simulink model "My_gfm_pv_plus_sil_motor"  (R2018b)
settings: Solver=ode45  StartTime=0.0  StopTime=22  RelTol=1e-3
PreLoadFcn:
  | lmodelDir = fileparts(get_param(bdroot,'FileName'));
  | 
  | load_system(fullfile(modelDir,'controls_element_lib.slx'));
  | load_system(fullfile(modelDir,'test_sequence_lib.slx'));
InitFcn:
  | close all;
  | clear all;
  | clc;
  | 
  | % frequency nominals
  | F_NOM = 60;
  | W_NOM = 2 * pi * F_NOM;
  | 
  | C_DC = 0.4; % Supercap: 0.5sec * 5MW
  | V_LVDC_NOM = 1000;
  | 
  | % base values relative to inverter
  | % --------------------------------
  | VLL_INV_NOM = 480;
  | P_INV_NOM = 1e6;
  | Q_INV_NOM = 0.5e6;
  | S_INV_NOM = sqrt(P_INV_NOM^2 + Q_INV_NOM^2);
  | 
  | I_INV_BASE = S_INV_NOM/(sqrt(3)*VLL_INV_NOM);
  | Z_INV_BASE = VLL_INV_NOM^2/S_INV_NOM;
  | L_INV_BASE = Z_INV_BASE / W_NOM;
  | C_INV_BASE = 1 / (Z_INV_BASE * W_NOM);
  | 
  | % nominal ratings for power system model
  | % --------------------------------------
  | INVERTER_COUNT = 100;
  | 
  | VLV_NOM = VLL_INV_NOM;
  | VMV_NOM = 35e3;
  | VHV_NOM = 230e3;
  | S_PLANT = INVERTER_COUNT * S_INV_NOM;
  | 
  | N_GSU = VHV_NOM/VMV_NOM;
  | N_MVT = VMV_NOM/VLV_NOM;
  | 
  | I_LV_BASE = S_PLANT/(sqrt(3)*VLV_NOM);
  | I_MV_BASE = S_PLANT/(sqrt(3)*VMV_NOM);
  | I_HV_BASE = S_PLANT/(sqrt(3)*VHV_NOM);
  | 
  | Z_LV_BASE = VLV_NOM^2/S_PLANT;
  | Z_MV_BASE = VMV_NOM^2/S_PLANT;
  | Z_HV_BASE = VHV_NOM^2/S_PLANT;
  | 
  | L_LV_BASE = Z_LV_BASE / W_NOM;
  | L_MV_BASE = Z_MV_BASE / W_NOM;
  | L_HV_BASE = Z_HV_BASE / W_NOM;
  | C_LV_BASE = 1 / (Z_LV_BASE * W_NOM);
  | C_MV_BASE = 1 / (Z_MV_BASE * W_NOM);
  | C_HV_BASE = 1 / (Z_HV_BASE * W_NOM);
  | 
  | %---------------------------------------
  | %Motor Control
  | 
  | Jsys = 20;
  | Fpu = 0.02;
  | MtrPwr = 500000 ;
  | MtrFreq = 60;
  | MtrPp = 2;
  | MtrWm = 2 * pi *MtrFreq/MtrPp;
  | MtrTrq = MtrPwr / MtrWm;
  | F = (Fpu*MtrTrq)/MtrWm;
  | 
  | SpeedBW = 2 * pi * 0.5;
  | Zeta = 1;
  | H = (0.5 * Jsys * MtrWm^2)/MtrPwr;
  | Kpv = SpeedBW * (H * 2) * 2 * Zeta;
  | Kiv = (SpeedBW^2) * (H * 2) * 1;
undefined symbols (not defined in the file): MtrNpFreq, MtrNpTrq, Pp, Ts_Control_1
libraries: test_sequence_lib x13, controls_element_lib x8, simulink x6
settings Model: SimulationMode=accelerator  Creator=halatrash  LastModifiedBy=ahhei
settings SolverCC: ZeroCrossAlgorithm=Adaptive
settings DataIOCC: ReturnWorkspaceOutputs=on
settings DebuggingCC: MaxConsecutiveZCsMsg=warning  IgnoredZcDiagnostic=none  UnconnectedInputMsg=none  UnconnectedOutputMsg=none  UnconnectedLineMsg=none
settings ModelReferenceCC: EnableRefExpFcnMdlSchedulingChecks=off
settings RTWCC: Description=Generic Real-Time Target

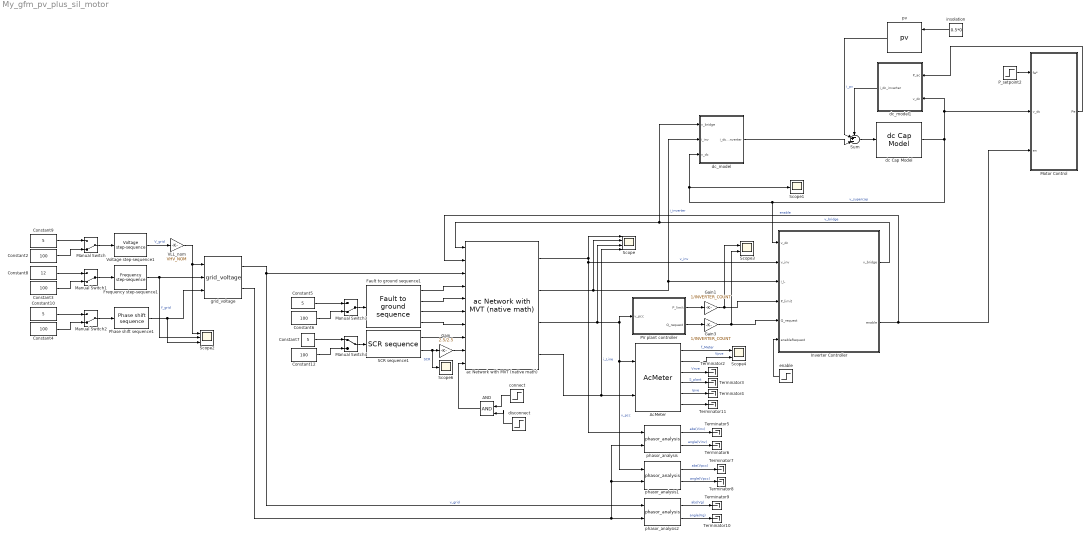
== system My_gfm_pv_plus_sil_motor ==
  AND : Logic  IconShape=distinctive  AllPortsSameDT=off  OutDataTypeStr=boolean
  AcMeter : test_sequence_lib/AcMeter  VllRated=VHV_NOM
  Constant{5,7,9..10} (4 alike) : Constant  Value=5
  Constant{2..4,6,12} (5 alike) : Constant  Value=100
  Constant8 : Constant  Value=12
  Fault to ground sequence1 : test_sequence_lib/Fault to ground sequence  SystemSampleTime=-1
  Frequency step-sequence1 : test_sequence_lib/Frequency step-sequence  SystemSampleTime=-1
  Gain : Gain  Gain=2.5/2.5
  Gain1 : Gain  Gain=1/INVERTER_COUNT
  Gain3 : Gain  Gain=1/INVERTER_COUNT
  Inverter Controller : Subsystem
  Manual Switch{,1..3} (4 alike) : ManualSwitch  CurrentSetting=0
  Manual Switch4 : ManualSwitch
  Motor Control : Subsystem
  PV plant controller : Subsystem  AncestorBlock=controls_element_lib/PV plant controller
  P_setpoint2 : Step  Time=4  SampleTime=0
  Phase shift sequence1 : test_sequence_lib/Phase shift sequence  SystemSampleTime=-1
  SCR sequence1 : test_sequence_lib/SCR sequence  SystemSampleTime=-1
  Scope : Scope  NumInputPorts=4
  Scope1 : Scope
  Scope2 : Scope  NumInputPorts=3
  Scope3 : Scope  NumInputPorts=2
  Scope4 : Scope  NumInputPorts=2
  Scope6 : Scope
  Sum : Sum  Inputs=-+-|
  Terminator{2..11} (10 alike) : Terminator
  VLL_nom : Gain  Gain=VHV_NOM
  Voltage step-sequence1 : test_sequence_lib/Voltage step-sequence  SystemSampleTime=-1
  ac Network with MVT (native math) : test_sequence_lib/ac Network with MVT (native math)  SystemSampleTime=-1
  connect : Step  Time=0  SampleTime=0
  dc Cap Model : test_sequence_lib/dc Cap Model  SystemSampleTime=-1
  dc_model : Subsystem  AncestorBlock=test_sequence_lib/dc_model
  dc_model1 : Subsystem  AncestorBlock=test_sequence_lib/dc_model
  disconnect : Step  Time=97  Before=1  After=0  SampleTime=0
  enable : Step  Time=2  SampleTime=0
  grid_voltage : test_sequence_lib/grid_voltage  SystemSampleTime=-1
  insolation : Constant  Value=0.5*0
  phasor_analysis : test_sequence_lib/phasor_analysis  SystemSampleTime=-1
  phasor_analysis1 : test_sequence_lib/phasor_analysis  SystemSampleTime=-1
  phasor_analysis2 : test_sequence_lib/phasor_analysis  SystemSampleTime=-1
  pv : test_sequence_lib/pv  VopenCircuit=1500  IshortCircuit=1000
  wires:
  ac Network with MVT (native math)/3 -> Scope/3, PV plant controller/1(v_pcc), phasor_analysis1/1, AcMeter/1  "v_pcc"
  Gain3/1 -> Scope3/2, Inverter Controller/5(Q_request)
  AcMeter/2 -> Scope4/2  "Vpve"
  phasor_analysis2/2 -> Terminator10/1  "angle(Vg)"
  phasor_analysis1/2 -> Terminator8/1  "angle(Vpcc)"
  AcMeter/5 -> Terminator4/1  "Ipve"
  phasor_analysis2/1 -> Terminator9/1  "abs(Vg)"
  Inverter Controller/1(v_bridge) -> ac Network with MVT (native math)/1, dc_model/1(v_bridge)  "v_bridge"
  phasor_analysis1/1 -> Terminator7/1  "abs(Vpcc)"
  grid_voltage/1 -> ac Network with MVT (native math)/3, phasor_analysis2/1  "v_grid"
  connect/1 -> AND/1
  dc Cap Model/1 -> dc_model1/2(v_dc), Motor Control/2(v_dc), Scope1/1, dc_model/3(v_dc), Inverter Controller/1(v_dc)  "v_supercap"
  AcMeter/4 -> Terminator3/1  "S_plant"
  Phase shift sequence1/1 -> Scope2/3, grid_voltage/3
  Frequency step-sequence1/1 -> Scope2/2, grid_voltage/2  "f_grid"
  phasor_analysis/1 -> Terminator5/1  "abs(Vinv)"
  AcMeter/3 -> Terminator2/1  "Vnve"
  phasor_analysis/2 -> Terminator6/1  "angle(Vinv)"
  Sum/1 -> dc Cap Model/1
  ac Network with MVT (native math)/1 -> Scope/1, Inverter Controller/2(v_inv), phasor_analysis/1  "v_inv"
  AND/1 -> ac Network with MVT (native math)/10
  AcMeter/6 -> Terminator11/1
  Voltage step-sequence1/1 -> VLL_nom/1  "V_grid"
  grid_voltage/2 -> phasor_analysis1/2, phasor_analysis/2, phasor_analysis2/2
  disconnect/1 -> AND/2
  ac Network with MVT (native math)/2 -> Scope/2, Inverter Controller/3(i_L), dc_model/2(i_inv)  "i_inverter"
  PV plant controller/2(Q_request) -> Gain3/1
  ac Network with MVT (native math)/4 -> Scope/4, AcMeter/2  "i_Line"
  dc_model/1(i_dc_inverter) -> Sum/3
  Inverter Controller/2(enable) -> Motor Control/3(en), ac Network with MVT (native math)/2  "enable"
  VLL_nom/1 -> Scope2/1, grid_voltage/1
  enable/1 -> Inverter Controller/6(enableRequest)
  insolation/1 -> pv/1
  pv/1 -> Sum/2  "i_pv"
  PV plant controller/1(P_limit) -> Gain1/1
  Gain1/1 -> Scope3/1, Inverter Controller/4(P_limit)
  AcMeter/1 -> Scope4/1  "f_Meter"
  Constant10/1 -> Manual Switch2/1
  Constant9/1 -> Manual Switch/1
  Constant4/1 -> Manual Switch2/2
  Constant8/1 -> Manual Switch1/1
  Manual Switch1/1 -> Frequency step-sequence1/1
  Manual Switch2/1 -> Phase shift sequence1/1
  Manual Switch/1 -> Voltage step-sequence1/1
  Constant3/1 -> Manual Switch1/2
  Constant2/1 -> Manual Switch/2
  Constant12/1 -> Manual Switch4/2
  Constant6/1 -> Manual Switch3/2
  Manual Switch4/1 -> SCR sequence1/1
  Constant5/1 -> Manual Switch3/1
  Manual Switch3/1 -> Fault to ground sequence1/1
  Fault to ground sequence1/4 -> ac Network with MVT (native math)/7
  SCR sequence1/2 -> Scope6/1, Gain/1  "SCR"
  Fault to ground sequence1/1 -> ac Network with MVT (native math)/4
  SCR sequence1/1 -> ac Network with MVT (native math)/8
  Constant7/1 -> Manual Switch4/1
  Fault to ground sequence1/3 -> ac Network with MVT (native math)/6
  Fault to ground sequence1/2 -> ac Network with MVT (native math)/5
  Gain/1 -> ac Network with MVT (native math)/9
  P_setpoint2/1 -> Motor Control/1(fe*)
  Motor Control/1(Pe) -> dc_model1/1(P_ac)
  dc_model1/1(i_dc_inverter) -> Sum/1

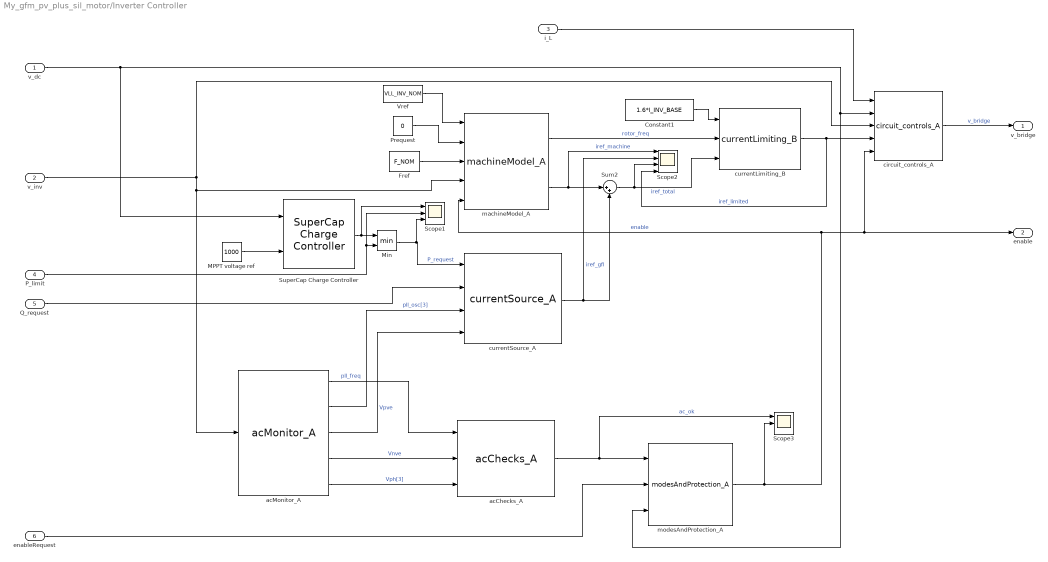
== system My_gfm_pv_plus_sil_motor/Inverter Controller ==
  v_dc : Inport
  v_inv : Inport  Port=2
  i_L : Inport  Port=3
  P_limit : Inport  Port=4
  Q_request : Inport  Port=5
  enableRequest : Inport  Port=6
  Constant1 : Constant  Value=1.6*I_INV_BASE
  Fref : Constant  Value=F_NOM
  MPPT voltage ref : Constant  Value=1000
  Min : MinMax  Inputs=2
  Prequest : Constant  Value=0
  Scope1 : Scope  NumInputPorts=3
  Scope2 : Scope  NumInputPorts=4
  Scope3 : Scope  NumInputPorts=3
  Sum2 : Sum  Inputs=|++
  SuperCap Charge Controller : controls_element_lib/SuperCap Charge Controller  SystemSampleTime=-1
  Vref : Constant  Value=VLL_INV_NOM
  acChecks_A : controls_element_lib/acChecks_A  VllRated=VLL_INV_NOM  nominalFrequency=F_NOM  tRequalify=2  T_CNTL=1e-3
  acMonitor_A : controls_element_lib/acMonitor_A  VllRated=VLL_INV_NOM  nominalFrequency=F_NOM
  circuit_controls_A : controls_element_lib/circuit_controls_A  SystemSampleTime=-1
  currentLimiting_B : controls_element_lib/currentLimiting_B  IRated=I_INV_BASE  peakSoftLimit=2.6  peakHardLimit=3.6
  currentSource_A : controls_element_lib/currentSource_A  VllRated=VLL_INV_NOM  SRated=S_INV_NOM  nominalFrequency=F_NOM  Plimit=P_INV_NOM/S_INV_NOM  Qlimit=Q_INV_NOM/S_INV_NOM
  machineModel_A : controls_element_lib/machineModel_A  SRated=S_INV_NOM  VllRated=VLL_INV_NOM  nominalFrequency=F_NOM  inertialConstant=0.1  kDroop=0  kDamper=0.5  Xs=0.3  rs=0.08  Qlimit=0.5  wExciter=10
  modesAndProtection_A : controls_element_lib/modesAndProtection_A  dcOvervotlageThreshold=1800  dcUndervotlageThreshold=700  dcTripClearTimeout=0.2
  v_bridge : Outport  VectorParamsAs1DForOutWhenUnconnected=on
  enable : Outport  Port=2  VectorParamsAs1DForOutWhenUnconnected=on
  wires:
  Vref/1 -> machineModel_A/1
  Prequest/1 -> machineModel_A/2
  Fref/1 -> machineModel_A/3
  machineModel_A/2 -> Scope2/1, Sum2/1  "iref_machine"
  currentLimiting_B/1 -> Scope2/4, circuit_controls_A/4  "iref_limited"
  v_inv/1 -> circuit_controls_A/3, acMonitor_A/1, machineModel_A/4
  currentSource_A/1 -> Scope2/2, Sum2/2  "iref_gfl"
  Sum2/1 -> Scope2/3, currentLimiting_B/3  "iref_total"
  acMonitor_A/2 -> currentSource_A/3  "pll_osc[3]"
  Q_request/1 -> currentSource_A/2
  acMonitor_A/4 -> acChecks_A/2  "Vnve"
  enableRequest/1 -> modesAndProtection_A/2
  modesAndProtection_A/1 -> Scope3/2, machineModel_A/5, circuit_controls_A/5, enable/1  "enable"
  Min/1 -> Scope1/3, currentSource_A/1  "P_request"
  acMonitor_A/3 -> currentSource_A/4  "Vpve"
  Constant1/1 -> currentLimiting_B/1
  acMonitor_A/5 -> acChecks_A/3  "Vph[3]"
  acChecks_A/1 -> Scope3/1, modesAndProtection_A/1  "ac_ok"
  acMonitor_A/1 -> acChecks_A/1  "pll_freq"
  circuit_controls_A/1 -> v_bridge/1  "v_bridge"
  v_dc/1 -> modesAndProtection_A/3, circuit_controls_A/2, SuperCap Charge Controller/1
  i_L/1 -> circuit_controls_A/1
  machineModel_A/1 -> currentLimiting_B/2  "rotor_freq"
  MPPT voltage ref/1 -> SuperCap Charge Controller/2
  SuperCap Charge Controller/1 -> Scope1/1, Min/1
  P_limit/1 -> Scope1/2, Min/2

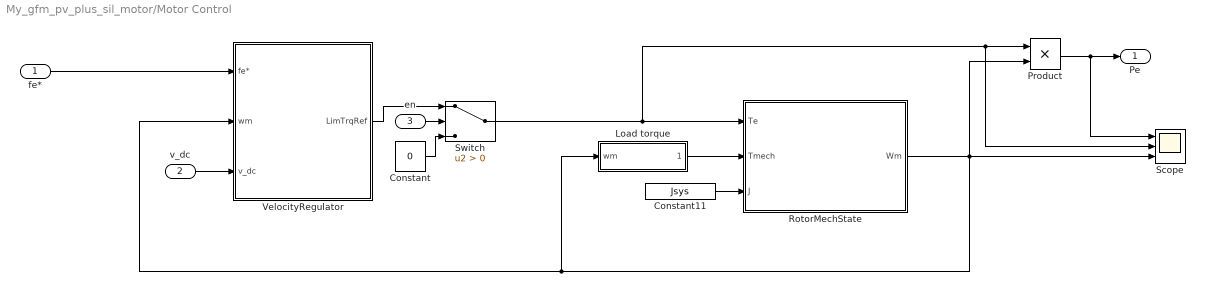
== system My_gfm_pv_plus_sil_motor/Motor Control ==
  fe* : Inport
  v_dc : Inport  Port=2
  en : Inport  Port=3
  Constant : Constant  Value=0
  Constant11 : Constant  Value=Jsys  OutDataTypeStr=double
  Load torque : Subsystem
  Product : Product
  RotorMechState : Subsystem
  Scope : Scope  NumInputPorts=3
  Switch : Switch  Criteria=u2 > Threshold
  VelocityRegulator : Subsystem
  Pe : Outport
  wires:
  RotorMechState/1(Wm) -> Product/2, Scope/3, VelocityRegulator/2(wm), Load torque/1(wm)
  Switch/1 -> Scope/2, Product/1, RotorMechState/1(Te)
  Constant11/1 -> RotorMechState/3(J)
  Load torque/1(" ") -> RotorMechState/2(Tmech)
  fe*/1 -> VelocityRegulator/1(fe*)
  Product/1 -> Scope/1, Pe/1
  v_dc/1 -> VelocityRegulator/3(v_dc)
  en/1 -> Switch/2
  VelocityRegulator/1(LimTrqRef) -> Switch/1
  Constant/1 -> Switch/3

== system My_gfm_pv_plus_sil_motor/PV plant controller ==
  v_pcc : Inport
  Frequency foldback : Subsystem
  Gain1 : Gain  Gain=S_PLANT
  Gain2 : Gain  Gain=S_PLANT
  Gain4 : Gain  Gain=1/VHV_NOM
  Meter : Subsystem
  VoltVAr : Subsystem
  P_limit : Outport  VectorParamsAs1DForOutWhenUnconnected=on
  Q_request : Outport  Port=2  VectorParamsAs1DForOutWhenUnconnected=on
  wires:
  Gain2/1 -> P_limit/1  "P_limit"
  Frequency foldback/1(limit_pu) -> Gain2/1
  Meter/1(f) -> Frequency foldback/1(f)
  v_pcc/1 -> Gain4/1
  Gain1/1 -> Q_request/1  "Q_request"
  Meter/2(V_estimate) -> VoltVAr/1(V)  "V_pu_plant"
  Gain4/1 -> Meter/1(v)
  VoltVAr/1(Q) -> Gain1/1

== system My_gfm_pv_plus_sil_motor/dc_model ==
  v_bridge : Inport
  i_inv : Inport  Port=2
  v_dc : Inport  Port=3
  Product : Product
  Product1 : Product  Inputs=*/
  Saturation : Saturate  UpperLimit=inf  LowerLimit=10
  Sum of Elements : Sum  Inputs=+
  i_dc_inverter : Outport  VectorParamsAs1DForOutWhenUnconnected=on
  wires:
  Saturation/1 -> Product1/2
  v_bridge/1 -> Product/1
  Product1/1 -> i_dc_inverter/1  "i_dc_inverter"
  Product/1 -> Sum of Elements/1
  i_inv/1 -> Product/2
  Sum of Elements/1 -> Product1/1  "P_ac"
  v_dc/1 -> Saturation/1

== system My_gfm_pv_plus_sil_motor/dc_model1 ==
  P_ac : Inport
  v_dc : Inport  Port=2
  Product1 : Product  Inputs=*/
  Saturation : Saturate  UpperLimit=inf  LowerLimit=10
  i_dc_inverter : Outport  VectorParamsAs1DForOutWhenUnconnected=on
  wires:
  Saturation/1 -> Product1/2
  Product1/1 -> i_dc_inverter/1
  P_ac/1 -> Product1/1
  v_dc/1 -> Saturation/1

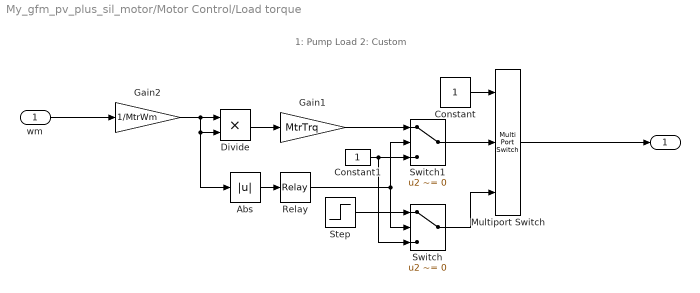
== system My_gfm_pv_plus_sil_motor/Motor Control/Load torque ==
  note: 1: Pump Load
      | 2: Custom
  wm : Inport
  Abs : Abs
  Constant : Constant
  Constant1 : Constant  OutDataTypeStr=single
  Divide : Product  Inputs=**
  Gain1 : Gain  Gain=MtrTrq
  Gain2 : Gain  Gain=1/MtrWm
  Multiport Switch : MultiPortSwitch  Inputs=2
  Relay : Relay  OnSwitchValue=0.01  OffSwitchValue=0.001
  Step : Step  Time=3  After=0.5*MtrTrq  SampleTime=0
  Switch : Switch  Criteria=u2 ~= 0
  Switch1 : Switch  Criteria=u2 ~= 0
  " " : Outport
  wires:
  Step/1 -> Switch/1
  Gain1/1 -> Switch1/1
  Constant/1 -> Multiport Switch/1
  Divide/1 -> Gain1/1
  wm/1 -> Gain2/1
  Switch/1 -> Multiport Switch/3
  Switch1/1 -> Multiport Switch/2
  Constant1/1 -> Switch/3, Switch1/3
  Relay/1 -> Switch1/2, Switch/2
  Abs/1 -> Relay/1
  Gain2/1 -> Abs/1, Divide/2, Divide/1
  Multiport Switch/1 -> " "/1

== system My_gfm_pv_plus_sil_motor/Motor Control/RotorMechState ==
  Te : Inport
  Tmech : Inport  Port=2
  J : Inport  Port=3
  Divide : Product  Inputs=*/
  Gain : Gain  Gain=F
  Integrator : Integrator
  Subtract : Sum  Inputs=-+-
  Wm : Outport
  wires:
  Te/1 -> Subtract/2
  Tmech/1 -> Subtract/3
  Subtract/1 -> Divide/1
  J/1 -> Divide/2
  Divide/1 -> Integrator/1
  Integrator/1 -> Gain/1, Wm/1
  Gain/1 -> Subtract/1

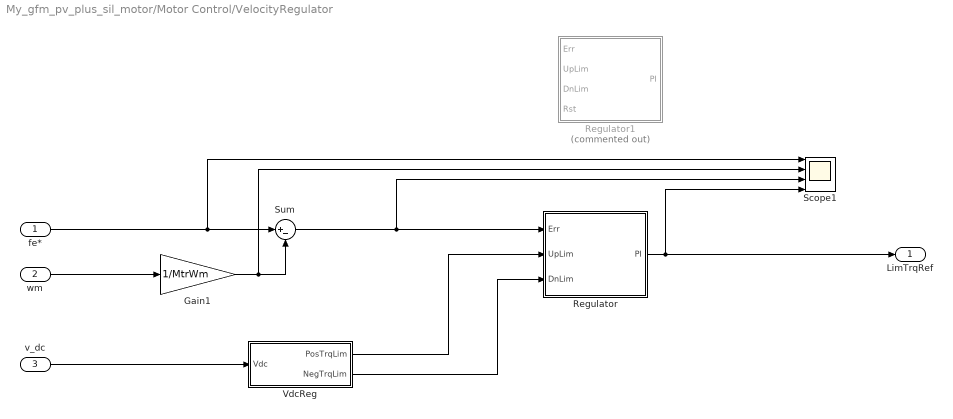
== system My_gfm_pv_plus_sil_motor/Motor Control/VelocityRegulator ==
  fe* : Inport
  wm : Inport  Port=2
  v_dc : Inport  Port=3
  Gain1 : Gain  Gain=1/MtrWm
  Regulator : Subsystem
  Regulator1 : Subsystem  Commented=on
  Scope1 : Scope  NumInputPorts=4
  Sum : Sum  Inputs=|+-
  VdcReg : Subsystem
  LimTrqRef : Outport
  wires:
  wm/1 -> Gain1/1
  v_dc/1 -> VdcReg/1(Vdc)
  Gain1/1 -> Scope1/2, Sum/2
  fe*/1 -> Scope1/1, Sum/1
  VdcReg/1(PosTrqLim) -> Regulator/2(UpLim)
  VdcReg/2(NegTrqLim) -> Regulator/3(DnLim)
  Regulator/1(PI) -> LimTrqRef/1, Scope1/4
  Sum/1 -> Regulator/1(Err), Scope1/3

== system My_gfm_pv_plus_sil_motor/PV plant controller/Frequency foldback ==
  f : Inport
  Constant : Constant  Value=F_NOM+0.5
  Gain : Gain  Gain=3
  Saturation : Saturate  UpperLimit=1  LowerLimit=0
  Sum : Sum  Inputs=|+-
  Transfer Fcn : TransferFcn  Denominator=[0.05 1]
  limit_pu : Outport  VectorParamsAs1DForOutWhenUnconnected=on
  wires:
  Saturation/1 -> limit_pu/1
  Constant/1 -> Sum/1
  Transfer Fcn/1 -> Gain/1
  Gain/1 -> Saturation/1
  f/1 -> Sum/2
  Sum/1 -> Transfer Fcn/1

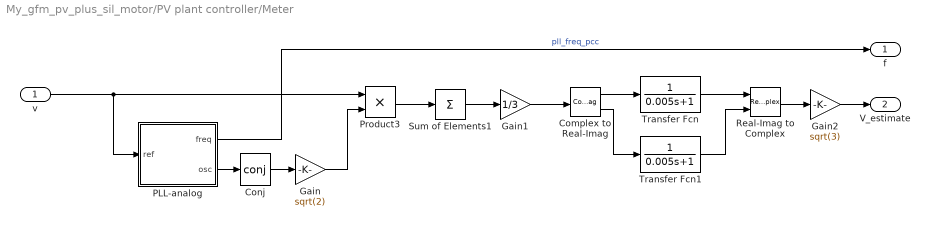
== system My_gfm_pv_plus_sil_motor/PV plant controller/Meter ==
  v : Inport
  Complex to Real-Imag : ComplexToRealImag
  Conj : Math  Operator=conj  SaturateOnIntegerOverflow=on
  Gain : Gain  Gain=sqrt(2)
  Gain1 : Gain  Gain=1/3
  Gain2 : Gain  Gain=sqrt(3)
  PLL-analog : Subsystem
  Product3 : Product
  Real-Imag to Complex : RealImagToComplex
  Sum of Elements1 : Sum  Inputs=+
  Transfer Fcn : TransferFcn  Denominator=[0.005 1]
  Transfer Fcn1 : TransferFcn  Denominator=[0.005 1]
  f : Outport  VectorParamsAs1DForOutWhenUnconnected=on
  V_estimate : Outport  Port=2  VectorParamsAs1DForOutWhenUnconnected=on
  wires:
  PLL-analog/1(freq) -> f/1  "pll_freq_pcc"
  Gain2/1 -> V_estimate/1
  Gain1/1 -> Complex to Real-Imag/1
  Gain/1 -> Product3/2
  Real-Imag to Complex/1 -> Gain2/1
  Conj/1 -> Gain/1
  PLL-analog/2(osc) -> Conj/1
  Complex to Real-Imag/1 -> Transfer Fcn/1
  v/1 -> Product3/1, PLL-analog/1(ref)
  Complex to Real-Imag/2 -> Transfer Fcn1/1
  Product3/1 -> Sum of Elements1/1
  Transfer Fcn/1 -> Real-Imag to Complex/1
  Sum of Elements1/1 -> Gain1/1
  Transfer Fcn1/1 -> Real-Imag to Complex/2

== system My_gfm_pv_plus_sil_motor/PV plant controller/VoltVAr ==
  V : Inport
  Abs : Abs
  Constant1 : Constant
  Gain : Gain  Gain=6
  Saturation : Saturate
  Sum1 : Sum  Inputs=|+-
  Transfer Fcn : TransferFcn  Denominator=[0.005 1]
  Q : Outport  VectorParamsAs1DForOutWhenUnconnected=on
  wires:
  Transfer Fcn/1 -> Q/1
  Saturation/1 -> Transfer Fcn/1
  V/1 -> Abs/1
  Abs/1 -> Sum1/2
  Constant1/1 -> Sum1/1
  Sum1/1 -> Gain/1
  Gain/1 -> Saturation/1

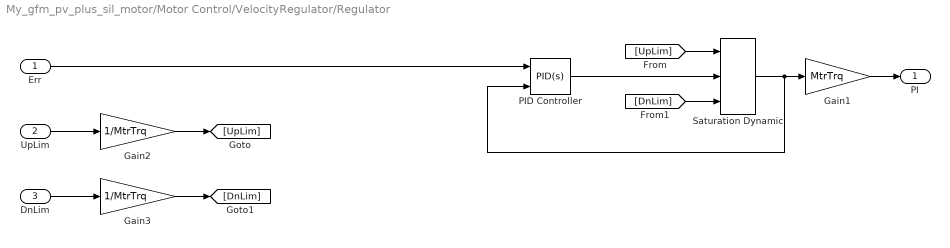
== system My_gfm_pv_plus_sil_motor/Motor Control/VelocityRegulator/Regulator ==
  Err : Inport
  UpLim : Inport  Port=2
  DnLim : Inport  Port=3
  Gain1 : Gain  Gain=MtrTrq
  Gain2 : Gain  Gain=1/MtrTrq
  Gain3 : Gain  Gain=1/MtrTrq
  PID Controller : simulink/Continuous/PID Controller  Controller=PID  Form=Parallel  TimeDomain=Continuous-time  SampleTime=-1  IntegratorMethod=Forward Euler  FilterMethod=Forward Euler  ControllerParametersSource=internal  P=Kpv  I=Kiv  D=0  UseFilter=on  N=100  TunerSelectOption=Transfer Function Based (PID Tuner App)  InitialConditionSource=internal  InitialConditionForIntegrator=0  InitialConditionForFilter=0  DifferentiatorICPrevScaledInput=0  ExternalReset=none  TrackingMode=on  Kt=1  LimitOutput=off  UpperSaturationLimit=inf  LowerSaturationLimit=-inf  LinearizeAsGain=on  AntiWindupMode=none  Kb=1  POutMin=[]  POutMax=[]  IOutMin=[]  IOutMax=[]  DOutMin=[]  DOutMax=[]  NOutMin=[]  NOutMax=[]  SumOutMin=[]  SumOutMax=[]  SaturationOutMin=[]  SaturationOutMax=[]  PParamMin=[]  PParamMax=[]  IParamMin=[]  IParamMax=[]  DParamMin=[]  DParamMax=[]  NParamMin=[]  NParamMax=[]  KbParamMin=[]  KbParamMax=[]  KtParamMin=[]  KtParamMax=[]  KbOutMin=[]  KbOutMax=[]  KtOutMin=[]  KtOutMax=[]  IntegratorOutMin=[]  IntegratorOutMax=[]  FilterOutMin=[]  FilterOutMax=[]  SumI1OutMin=[]  SumI1OutMax=[]  SumI2OutMin=[]  SumI2OutMax=[]  SumI3OutMin=[]  SumI3OutMax=[]  SumI4OutMin=[]  SumI4OutMax=[]  SumDOutMin=[]  SumDOutMax=[]  DifferentiatorOutMin=[]  DifferentiatorOutMax=[]  FilterDiffOutCoefMin=[]  FilterDiffOutCoefMax=[]  ReciprocalOutMin=[]  ReciprocalOutMax=[]  SumDenOutMin=[]  SumDenOutMax=[]  SumNumOutMin=[]  SumNumOutMax=[]  DivideOutMin=[]  DivideOutMax=[]  IntegratorContinuousStateAttributes=''  IntegratorStateMustResolveToSignalObject=off  IntegratorRTWStateStorageClass=Auto  FilterContinuousStateAttributes=''  FilterStateMustResolveToSignalObject=off  FilterRTWStateStorageClass=Auto  ParallelPVariant=InternalParameters  IdealPVariant=Disabled  IVariant=InternalParameters  DVariant=InternalParameters  IntegratorVariant=Continuous  SatVariant=Disabled  AWVariant=Passthrough  PCopyVariant=Disabled  TRVariant=Enabled  FdbkBlocksVariant=Forward  IdealPFdbkVariant=Disabled  SatFdbkVariant=Disabled  DerivativeFilterVariant=ContFilter  NVariant=InternalParameters  NCopyVariant=Disabled  FilterICVariant=InternalICsFilter  IntegratorICVariant=InternalICs  ExternalResetVariant=Disabled  TRSumVariant=TrackingMode  SumFdbkVariant=Disabled  SumVariant=Sum_PID
  Saturation Dynamic : simulink/Discontinuities/Saturation Dynamic  OutMin=[]  OutMax=[]  OutDataTypeStr=Inherit: Same as second input  OutDataType=fixdt(1, 16)  OutScaling=2^-10  DoSatur=off
  PI : Outport
  wires:
  UpLim/1 -> Gain2/1
  DnLim/1 -> Gain3/1
  Saturation Dynamic/1 -> PID Controller/2, Gain1/1
  Gain1/1 -> PI/1
  Gain2/1 -> [UpLim]
  Gain3/1 -> [DnLim]
  Err/1 -> PID Controller/1
  PID Controller/1 -> Saturation Dynamic/2
  [UpLim] -> Saturation Dynamic/1
  [DnLim] -> Saturation Dynamic/3

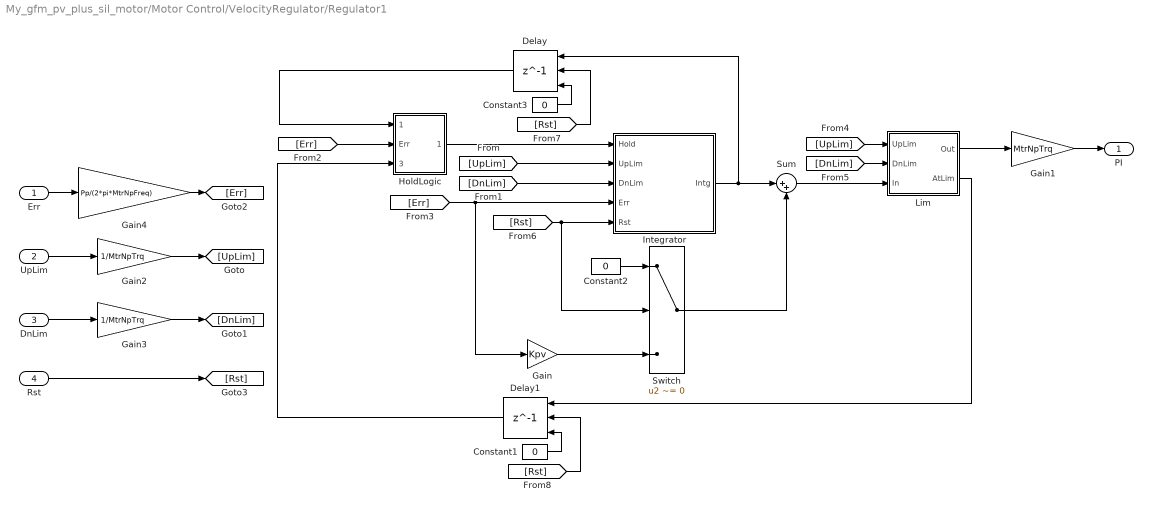
== system My_gfm_pv_plus_sil_motor/Motor Control/VelocityRegulator/Regulator1 ==
  Err : Inport
  UpLim : Inport  Port=2
  DnLim : Inport  Port=3
  Rst : Inport  Port=4
  Constant1 : Constant  Value=0  OutDataTypeStr=boolean
  Constant2 : Constant  Value=0  OutDataTypeStr=single
  Constant3 : Constant  Value=0  OutDataTypeStr=single
  Delay : Delay  DelayLength=1  InitialConditionSource=Input port  InitialCondition=0  ExternalReset=Rising
      settings: InputPortMap=u0,r5,p4
  Delay1 : Delay  DelayLength=1  InitialConditionSource=Input port  InitialCondition=0  ExternalReset=Rising
      settings: InputPortMap=u0,r5,p4
  Gain : Gain  Gain=Kpv
  Gain1 : Gain  Gain=MtrNpTrq
  Gain2 : Gain  Gain=1/MtrNpTrq
  Gain3 : Gain  Gain=1/MtrNpTrq
  Gain4 : Gain  Gain=Pp/(2*pi*MtrNpFreq)
  HoldLogic : Subsystem
  Integrator : Subsystem
  Lim : Subsystem
  Sum : Sum  Inputs=|++
  Switch : Switch  Criteria=u2 ~= 0
  PI : Outport
  wires:
  UpLim/1 -> Gain2/1
  DnLim/1 -> Gain3/1
  [UpLim] -> Integrator/2(UpLim)
  [DnLim] -> Integrator/3(DnLim)
  HoldLogic/1(Hold) -> Integrator/1(Hold)
  [Err] -> HoldLogic/2(Err)
  [Err] -> Integrator/4(Err), Gain/1
  Integrator/1(Intg) -> Delay/1, Sum/1
  Delay/1 -> HoldLogic/1(PrevOut)
  Sum/1 -> Lim/3(In)
  Lim/2(AtLim) -> Delay1/1
  Delay1/1 -> HoldLogic/3(AtLim)
  [UpLim] -> Lim/1(UpLim)
  [DnLim] -> Lim/2(DnLim)
  Rst/1 -> [Rst]
  Constant3/1 -> Delay/3
  [Rst] -> Delay/2
  [Rst] -> Delay1/2
  Constant1/1 -> Delay1/3
  [Rst] -> Switch/2, Integrator/5(Rst)
  Switch/1 -> Sum/2
  Gain/1 -> Switch/3
  Constant2/1 -> Switch/1
  Lim/1(Out) -> Gain1/1
  Gain1/1 -> PI/1
  Gain2/1 -> [UpLim]
  Gain3/1 -> [DnLim]
  Err/1 -> Gain4/1
  Gain4/1 -> [Err]

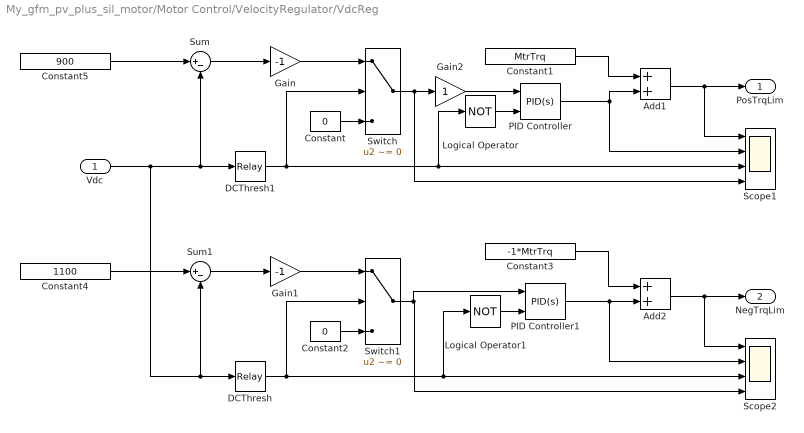
== system My_gfm_pv_plus_sil_motor/Motor Control/VelocityRegulator/VdcReg ==
  Vdc : Inport
  Add1 : Sum
  Add2 : Sum
  Constant : Constant  Value=0  OutDataTypeStr=single
  Constant1 : Constant  Value=MtrTrq  OutDataTypeStr=single
  Constant2 : Constant  Value=0  OutDataTypeStr=single
  Constant3 : Constant  Value=-1*MtrTrq  OutDataTypeStr=single
  Constant4 : Constant  Value=1100  OutDataTypeStr=single
  Constant5 : Constant  Value=900  OutDataTypeStr=single
  DCThresh : Relay  OnSwitchValue=1100  OffSwitchValue=1050
  DCThresh1 : Relay  OnSwitchValue=950  OffSwitchValue=900  OnOutputValue=0  OffOutputValue=1
  Gain : Gain  Gain=-1
  Gain1 : Gain  Gain=-1
  Gain2 : Gain
  Logical Operator : Logic  Operator=NOT  AllPortsSameDT=off  OutDataTypeStr=boolean
  Logical Operator1 : Logic  Operator=NOT  AllPortsSameDT=off  OutDataTypeStr=boolean
  PID Controller : simulink/Continuous/PID Controller  Controller=PID  Form=Parallel  TimeDomain=Continuous-time  SampleTime=-1  IntegratorMethod=Forward Euler  FilterMethod=Forward Euler  ControllerParametersSource=internal  P=100  I=200  D=0  UseFilter=on  N=100  TunerSelectOption=Transfer Function Based (PID Tuner App)  InitialConditionSource=internal  InitialConditionForIntegrator=0  InitialConditionForFilter=0  DifferentiatorICPrevScaledInput=0  ExternalReset=level  TrackingMode=off  Kt=1  LimitOutput=on  UpperSaturationLimit=0  LowerSaturationLimit=-2*MtrTrq  LinearizeAsGain=on  AntiWindupMode=clamping  Kb=1  POutMin=[]  POutMax=[]  IOutMin=[]  IOutMax=[]  DOutMin=[]  DOutMax=[]  NOutMin=[]  NOutMax=[]  SumOutMin=[]  SumOutMax=[]  SaturationOutMin=[]  SaturationOutMax=[]  PParamMin=[]  PParamMax=[]  IParamMin=[]  IParamMax=[]  DParamMin=[]  DParamMax=[]  NParamMin=[]  NParamMax=[]  KbParamMin=[]  KbParamMax=[]  KtParamMin=[]  KtParamMax=[]  KbOutMin=[]  KbOutMax=[]  KtOutMin=[]  KtOutMax=[]  IntegratorOutMin=[]  IntegratorOutMax=[]  FilterOutMin=[]  FilterOutMax=[]  SumI1OutMin=[]  SumI1OutMax=[]  SumI2OutMin=[]  SumI2OutMax=[]  SumI3OutMin=[]  SumI3OutMax=[]  SumI4OutMin=[]  SumI4OutMax=[]  SumDOutMin=[]  SumDOutMax=[]  DifferentiatorOutMin=[]  DifferentiatorOutMax=[]  FilterDiffOutCoefMin=[]  FilterDiffOutCoefMax=[]  ReciprocalOutMin=[]  ReciprocalOutMax=[]  SumDenOutMin=[]  SumDenOutMax=[]  SumNumOutMin=[]  SumNumOutMax=[]  DivideOutMin=[]  DivideOutMax=[]  IntegratorContinuousStateAttributes=''  IntegratorStateMustResolveToSignalObject=off  IntegratorRTWStateStorageClass=Auto  FilterContinuousStateAttributes=''  FilterStateMustResolveToSignalObject=off  FilterRTWStateStorageClass=Auto  ParallelPVariant=InternalParameters  IdealPVariant=Disabled  IVariant=InternalParameters  DVariant=InternalParameters  IntegratorVariant=Continuous  SatVariant=Enabled  AWVariant=ContClampingParallel  PCopyVariant=Disabled  TRVariant=Disabled  FdbkBlocksVariant=Forward  IdealPFdbkVariant=Disabled  SatFdbkVariant=Disabled  DerivativeFilterVariant=ContFilter  NVariant=InternalParameters  NCopyVariant=Disabled  FilterICVariant=InternalICsFilter  IntegratorICVariant=InternalICs  ExternalResetVariant=ExternalReset  TRSumVariant=Passthrough  SumFdbkVariant=Disabled  SumVariant=Sum_PID
  PID Controller1 : simulink/Continuous/PID Controller  Controller=PID  Form=Parallel  TimeDomain=Continuous-time  SampleTime=-1  IntegratorMethod=Forward Euler  FilterMethod=Forward Euler  ControllerParametersSource=internal  P=100  I=200  D=0  UseFilter=on  N=100  TunerSelectOption=Transfer Function Based (PID Tuner App)  InitialConditionSource=internal  InitialConditionForIntegrator=0  InitialConditionForFilter=0  DifferentiatorICPrevScaledInput=0  ExternalReset=level  TrackingMode=off  Kt=1  LimitOutput=on  UpperSaturationLimit=2*MtrTrq  LowerSaturationLimit=0  LinearizeAsGain=on  AntiWindupMode=clamping  Kb=1  POutMin=[]  POutMax=[]  IOutMin=[]  IOutMax=[]  DOutMin=[]  DOutMax=[]  NOutMin=[]  NOutMax=[]  SumOutMin=[]  SumOutMax=[]  SaturationOutMin=[]  SaturationOutMax=[]  PParamMin=[]  PParamMax=[]  IParamMin=[]  IParamMax=[]  DParamMin=[]  DParamMax=[]  NParamMin=[]  NParamMax=[]  KbParamMin=[]  KbParamMax=[]  KtParamMin=[]  KtParamMax=[]  KbOutMin=[]  KbOutMax=[]  KtOutMin=[]  KtOutMax=[]  IntegratorOutMin=[]  IntegratorOutMax=[]  FilterOutMin=[]  FilterOutMax=[]  SumI1OutMin=[]  SumI1OutMax=[]  SumI2OutMin=[]  SumI2OutMax=[]  SumI3OutMin=[]  SumI3OutMax=[]  SumI4OutMin=[]  SumI4OutMax=[]  SumDOutMin=[]  SumDOutMax=[]  DifferentiatorOutMin=[]  DifferentiatorOutMax=[]  FilterDiffOutCoefMin=[]  FilterDiffOutCoefMax=[]  ReciprocalOutMin=[]  ReciprocalOutMax=[]  SumDenOutMin=[]  SumDenOutMax=[]  SumNumOutMin=[]  SumNumOutMax=[]  DivideOutMin=[]  DivideOutMax=[]  IntegratorContinuousStateAttributes=''  IntegratorStateMustResolveToSignalObject=off  IntegratorRTWStateStorageClass=Auto  FilterContinuousStateAttributes=''  FilterStateMustResolveToSignalObject=off  FilterRTWStateStorageClass=Auto  ParallelPVariant=InternalParameters  IdealPVariant=Disabled  IVariant=InternalParameters  DVariant=InternalParameters  IntegratorVariant=Continuous  SatVariant=Enabled  AWVariant=ContClampingParallel  PCopyVariant=Disabled  TRVariant=Disabled  FdbkBlocksVariant=Forward  IdealPFdbkVariant=Disabled  SatFdbkVariant=Disabled  DerivativeFilterVariant=ContFilter  NVariant=InternalParameters  NCopyVariant=Disabled  FilterICVariant=InternalICsFilter  IntegratorICVariant=InternalICs  ExternalResetVariant=ExternalReset  TRSumVariant=Passthrough  SumFdbkVariant=Disabled  SumVariant=Sum_PID
  Scope1 : Scope  NumInputPorts=4
  Scope2 : Scope  NumInputPorts=4
  Sum : Sum  Inputs=|+-
  Sum1 : Sum  Inputs=|+-
  Switch : Switch  Criteria=u2 ~= 0
  Switch1 : Switch  Criteria=u2 ~= 0
  PosTrqLim : Outport
  NegTrqLim : Outport  Port=2
  wires:
  Sum/1 -> Gain/1
  Gain/1 -> Switch/1
  Constant/1 -> Switch/3
  PID Controller/1 -> Add1/2, Scope1/2
  Constant1/1 -> Add1/1
  Add1/1 -> Scope1/1, PosTrqLim/1
  Switch/1 -> Gain2/1, Scope1/4
  Constant3/1 -> Add2/1
  Add2/1 -> Scope2/1, NegTrqLim/1
  PID Controller1/1 -> Add2/2, Scope2/2
  Constant2/1 -> Switch1/3
  Sum1/1 -> Gain1/1
  Vdc/1 -> DCThresh/1, Sum1/2, DCThresh1/1, Sum/2
  Constant5/1 -> Sum/1
  Gain1/1 -> Switch1/1
  Constant4/1 -> Sum1/1
  Logical Operator/1 -> PID Controller/2
  DCThresh1/1 -> Switch/2, Logical Operator/1, Scope1/3
  Logical Operator1/1 -> PID Controller1/2
  Switch1/1 -> PID Controller1/1, Scope2/4
  DCThresh/1 -> Switch1/2, Logical Operator1/1, Scope2/3
  Gain2/1 -> PID Controller/1

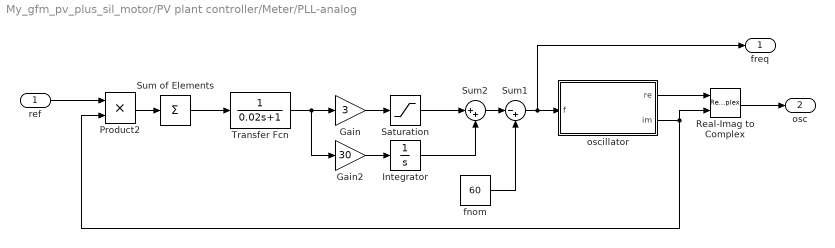
== system My_gfm_pv_plus_sil_motor/PV plant controller/Meter/PLL-analog ==
  ref : Inport
  Gain : Gain  Gain=3
  Gain2 : Gain  Gain=30
  Integrator : Integrator  LimitOutput=on  UpperSaturationLimit=5  LowerSaturationLimit=-5
  Product2 : Product
  Real-Imag to Complex : RealImagToComplex
  Saturation : Saturate  UpperLimit=5  LowerLimit=-5
  Sum of Elements : Sum  Inputs=+
  Sum1 : Sum  Inputs=|-+
  Sum2 : Sum  Inputs=|++
  Transfer Fcn : TransferFcn  Denominator=[0.02 1]
  fnom : Constant  Value=60
  oscillator : Subsystem
  freq : Outport  VectorParamsAs1DForOutWhenUnconnected=on
  osc : Outport  Port=2  VectorParamsAs1DForOutWhenUnconnected=on
  wires:
  Gain2/1 -> Integrator/1
  Integrator/1 -> Sum2/2
  Sum2/1 -> Sum1/1
  fnom/1 -> Sum1/2
  Product2/1 -> Sum of Elements/1
  oscillator/2(im) -> Product2/2, Real-Imag to Complex/2
  Transfer Fcn/1 -> Gain/1, Gain2/1
  Saturation/1 -> Sum2/1
  Gain/1 -> Saturation/1
  Sum1/1 -> freq/1, oscillator/1(f)
  ref/1 -> Product2/1
  oscillator/1(re) -> Real-Imag to Complex/1
  Real-Imag to Complex/1 -> osc/1
  Sum of Elements/1 -> Transfer Fcn/1

== system My_gfm_pv_plus_sil_motor/Motor Control/VelocityRegulator/Regulator1/HoldLogic ==
  PrevOut : Inport
  Err : Inport  Port=2
  AtLim : Inport  Port=3
  Compare To Zero : simulink/Logic and Bit Operations/Compare To Zero  relop=>=  OutDataTypeStr=boolean
  Logical Operator : Logic  AllPortsSameDT=off  OutDataTypeStr=boolean
  Product : Product
  Sign : Signum
  Sign1 : Signum
  Hold : Outport
  wires:
  PrevOut/1 -> Sign/1
  Err/1 -> Sign1/1
  Sign/1 -> Product/1
  Sign1/1 -> Product/2
  Product/1 -> Compare To Zero/1
  Compare To Zero/1 -> Logical Operator/1
  Logical Operator/1 -> Hold/1
  AtLim/1 -> Logical Operator/2

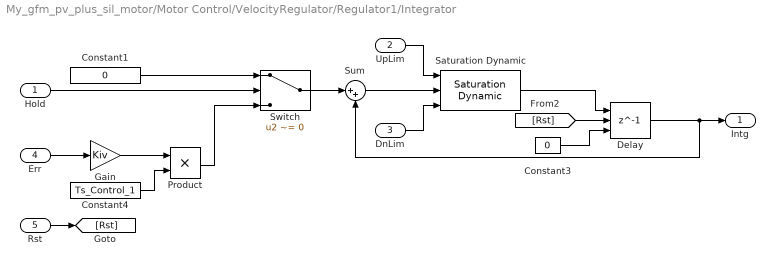
== system My_gfm_pv_plus_sil_motor/Motor Control/VelocityRegulator/Regulator1/Integrator ==
  Hold : Inport
  UpLim : Inport  Port=2
  DnLim : Inport  Port=3
  Err : Inport  Port=4
  Rst : Inport  Port=5
  Constant1 : Constant  Value=0  OutDataTypeStr=single
  Constant3 : Constant  Value=0  OutDataTypeStr=single
  Constant4 : Constant  Value=Ts_Control_1  OutDataTypeStr=single
  Delay : Delay  DelayLength=1  InitialConditionSource=Input port  InitialCondition=0  ExternalReset=Rising
      settings: InputPortMap=u0,r5,p4
  Gain : Gain  Gain=Kiv
  Product : Product
  Saturation Dynamic : simulink/Discontinuities/Saturation Dynamic  OutMin=[]  OutMax=[]  OutDataTypeStr=Inherit: Same as second input  OutDataType=fixdt(1, 16)  OutScaling=2^-10  DoSatur=off
  Sum : Sum  Inputs=|++
  Switch : Switch  Criteria=u2 ~= 0
  Intg : Outport
  wires:
  Hold/1 -> Switch/2
  Delay/1 -> Sum/2, Intg/1
  Switch/1 -> Sum/1
  Sum/1 -> Saturation Dynamic/2
  UpLim/1 -> Saturation Dynamic/1
  DnLim/1 -> Saturation Dynamic/3
  Err/1 -> Gain/1
  Gain/1 -> Product/1
  Product/1 -> Switch/3
  Constant4/1 -> Product/2
  Constant1/1 -> Switch/1
  Constant3/1 -> Delay/3
  Saturation Dynamic/1 -> Delay/1
  [Rst] -> Delay/2
  Rst/1 -> [Rst]

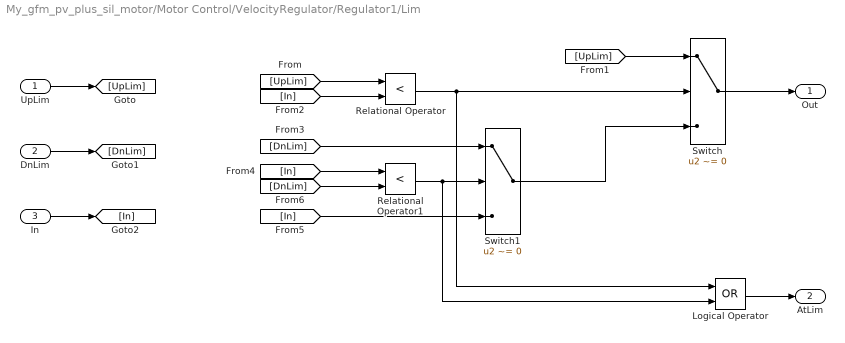
== system My_gfm_pv_plus_sil_motor/Motor Control/VelocityRegulator/Regulator1/Lim ==
  UpLim : Inport
  DnLim : Inport  Port=2
  In : Inport  Port=3
  Logical Operator : Logic  Operator=OR  AllPortsSameDT=off  OutDataTypeStr=boolean
  Relational Operator : RelationalOperator  Operator=<  OutDataTypeStr=boolean  RndMeth=Simplest
  Relational Operator1 : RelationalOperator  Operator=<  OutDataTypeStr=boolean  RndMeth=Simplest
  Switch : Switch  Criteria=u2 ~= 0
  Switch1 : Switch  Criteria=u2 ~= 0
  Out : Outport
  AtLim : Outport  Port=2
  wires:
  [UpLim] -> Relational Operator/1
  Relational Operator/1 -> Logical Operator/1, Switch/2
  Switch/1 -> Out/1
  Relational Operator1/1 -> Logical Operator/2, Switch1/2
  Switch1/1 -> Switch/3
  Logical Operator/1 -> AtLim/1
  UpLim/1 -> [UpLim]
  DnLim/1 -> [DnLim]
  [UpLim] -> Switch/1
  In/1 -> [In]
  [In] -> Relational Operator/2
  [DnLim] -> Switch1/1
  [In] -> Relational Operator1/1
  [In] -> Switch1/3
  [DnLim] -> Relational Operator1/2

== system My_gfm_pv_plus_sil_motor/PV plant controller/Meter/PLL-analog/oscillator ==
  f : Inport
  2*pi : Gain  Gain=2*pi
  Cos : Trigonometry  Operator=cos
  Integrator : Integrator
  Rotation : Constant  Value=[0 -1 -2]*1/3
  Sin : Trigonometry
  Sum : Sum  Inputs=|++
  re : Outport  VectorParamsAs1DForOutWhenUnconnected=on
  im : Outport  Port=2  VectorParamsAs1DForOutWhenUnconnected=on
  wires:
  2*pi/1 -> Sin/1, Cos/1
  f/1 -> Integrator/1
  Cos/1 -> re/1
  Sin/1 -> im/1
  Sum/1 -> 2*pi/1
  Integrator/1 -> Sum/1
  Rotation/1 -> Sum/2
